simulink model "Filtertianzy17"  (R2019a)
settings: Solver=FixedStepAuto  StartTime=0.0  StopTime=2  FixedStep=0.01  RelTol=1e-3
InitFcn:
  | a=10*ones(1,50);
  | b=8*ones(1,50);
  | c=-8*ones(1,3);
  | d=8*ones(1,50);
  | tzy=[a b c d];
libraries: dspsrcs4 x1
settings Model: Creator=dell  LastModifiedBy=MSI1
settings DataIOCC: ReturnWorkspaceOutputs=off
settings DebuggingCC: ArithmeticOperatorsInVariantConditions=warning

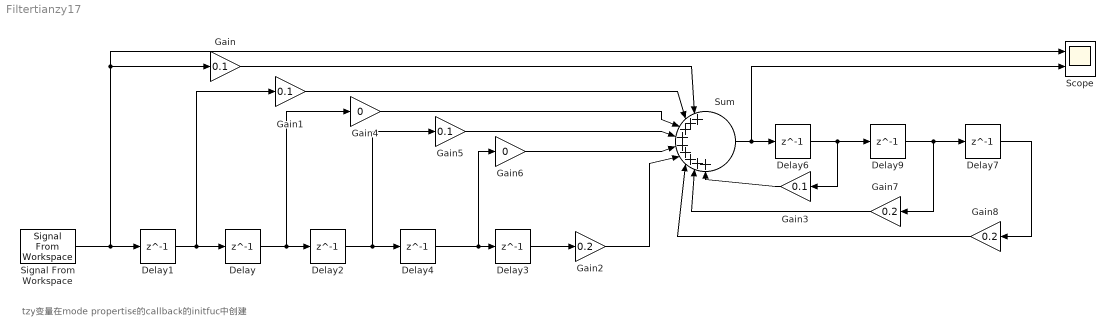
== system Filtertianzy17 ==
  note: tzy变量在mode propertise的callback的initfuc中创建
  Delay{,1..4,6..7,9} (8 alike) : Delay  DelayLength=1  InitialCondition=0
  Gain{,1,3,5} (4 alike) : Gain  Gain=0.1
  Gain2 : Gain  Gain=0.2
  Gain4 : Gain  Gain=0
  Gain6 : Gain  Gain=0
  Gain7 : Gain  Gain=0.2
  Gain8 : Gain  Gain=0.2
  Scope : Scope  NumInputPorts=2
  Signal From Workspace : dspsrcs4/Signal From Workspace  X=tzy  Ts=0.01  nsamps=1  OutputAfterFinalValue=Setting to zero  ignoreOrWarnInputAndFrameLengths=off  OutputFrames=off
  Sum : Sum  Inputs=|+++++++++
  wires:
  Delay1/1 -> Delay/1, Gain1/1
  Delay/1 -> Gain4/1, Delay2/1
  Delay2/1 -> Gain5/1, Delay4/1
  Delay4/1 -> Gain6/1, Delay3/1
  Delay3/1 -> Gain2/1
  Delay6/1 -> Gain3/1, Delay9/1
  Delay9/1 -> Gain7/1, Delay7/1
  Delay7/1 -> Gain8/1
  Gain/1 -> Sum/1
  Gain1/1 -> Sum/2
  Gain4/1 -> Sum/3
  Gain5/1 -> Sum/4
  Gain6/1 -> Sum/5
  Gain2/1 -> Sum/6
  Signal From Workspace/1 -> Scope/1, Gain/1, Delay1/1
  Sum/1 -> Scope/2, Delay6/1
  Gain3/1 -> Sum/9
  Gain7/1 -> Sum/8
  Gain8/1 -> Sum/7
